simulink model "Control"  (R2023b)
settings: Solver=VariableStepAuto  StartTime=0.0  StopTime=0.5  RelTol=1e-3
values from neighbouring files (symbols this model uses):
  f_v = 1.7086e-04    (= 0.00017086)    [Control0.m]
  i = 12    [Control0.m]    (also in Electromechanical_coupling0.m; Figure3_9.m; Figure4_1819.m)
  J = J_m+J_eq+J_L/(i^2)    (= 0.000140202493333)    [Control0.m]    (also in Electromechanical_coupling0.m; Figure3_9.m = 0.000114299715556)
  J_eq = 3.53416e-6    (= 3.53416e-06)    [Control0.m]    (also in Electromechanical_coupling0.m)
  J_L = 4530e-6    (= 0.00453)    [Control0.m]    (also in Electromechanical_coupling0.m)
  J_m = 105.21e-6    (= 0.00010521)    [Control0.m]    (also in Electromechanical_coupling0.m)
  J_total = J_m+J_eq+(1/(i^2)+miu/i)*J_L    (= 0.000143184743333)    [Control0.m]
  Jeq = 3.53416e-6    (= 3.53416e-06)    [Figure3_9.m]    (also in Figure4_1819.m = 0.000143184743333)
  JL = 800e-6    (= 0.0008)    [Figure3_9.m]    (also in Figure4_1819.m = 0.00453)
  Jm = 105.21e-6    (= 0.00010521)    [Figure3_9.m]    (also in Figure4_1819.m)
  K_t = 3/2 * P_n * phi_f    (= 0.28077)    [Control0.m]    (also in Electromechanical_coupling0.m)
  Kic = 2000    [Control0.m]    (also in Figure3_9.m)
  Kic_2 = R_s/L_q    (= 719.178082192)    [Control0.m]
  Kis = 10    [Control0.m]    (also in Figure3_9.m = 20)
  Kis_2 = 1/(3*TPWM*delta^2)    (= 92.5925925926)    [Control0.m]
  Kpc = 3    [Control0.m]    (also in Figure3_9.m)
  Kpc_2 = L_q/(3*TPWM)    (= 4.86666666667)    [Control0.m]
  Kps = 0.15    [Control0.m]    (also in Figure3_9.m = 0.2)
  Kps_2 = J_total/(3*TPWM*delta*K_t)    (= 0.283317589592)    [Control0.m]
  Kt = 3/2 * Pn * Flux    (= 0.28077)    [Figure3_9.m]    (also in Figure4_1819.m)
  L_d = 1.46e-3    (= 0.00146)    [Control0.m]    (also in Electromechanical_coupling0.m)
  L_q = L_d    (= 0.00146)    [Control0.m]    (also in Electromechanical_coupling0.m)
  miu = 0.0079    [Control0.m]    (also in Figure4_1819.m)
  NtoW = pi / 30    (= 0.10471975512)    [Control0.m]    (also in Electromechanical_coupling0.m)
  P_n = 14    [Control0.m]    (also in Electromechanical_coupling0.m)
  phi_f = 0.01337    [Control0.m]    (also in Electromechanical_coupling0.m)
  R_s = 1.05    [Control0.m]    (also in Electromechanical_coupling0.m)
  T_c0 = 0.0104    [Control0.m]
  TPWM = 1/10000    (= 0.0001)    [Control0.m]
  U_dc = 72    [Control0.m]
  WtoN = 30 / pi    (= 9.54929658551)    [Control0.m]    (also in Electromechanical_coupling0.m)
undefined symbols (not defined in the file or in its folder): fv, Tc0
libraries: spsStairGeneratorLib x20, slpidlib x15, spsDCVoltageSourceLib x5, spsUniversalBridgeLib x5, spsPermanentMagnetSynchronousMachineLib x5, spsSVPWMGenerator2LevelLib x5, sps_lib x1, simulink x1
(part 1 of 3)
settings Model: Creator=Administrator  LastModifiedBy=Administrator

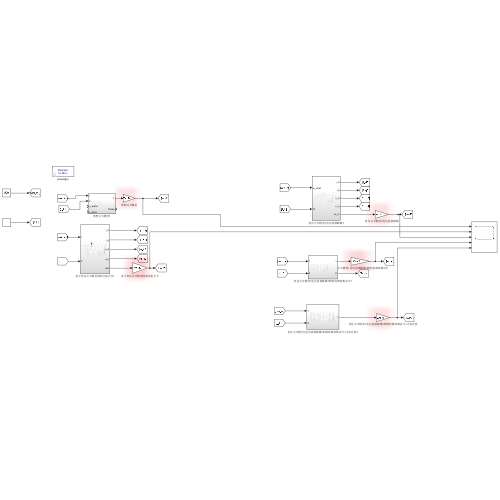
[thumbnail: Simulink's stored preview of the top-level diagram]
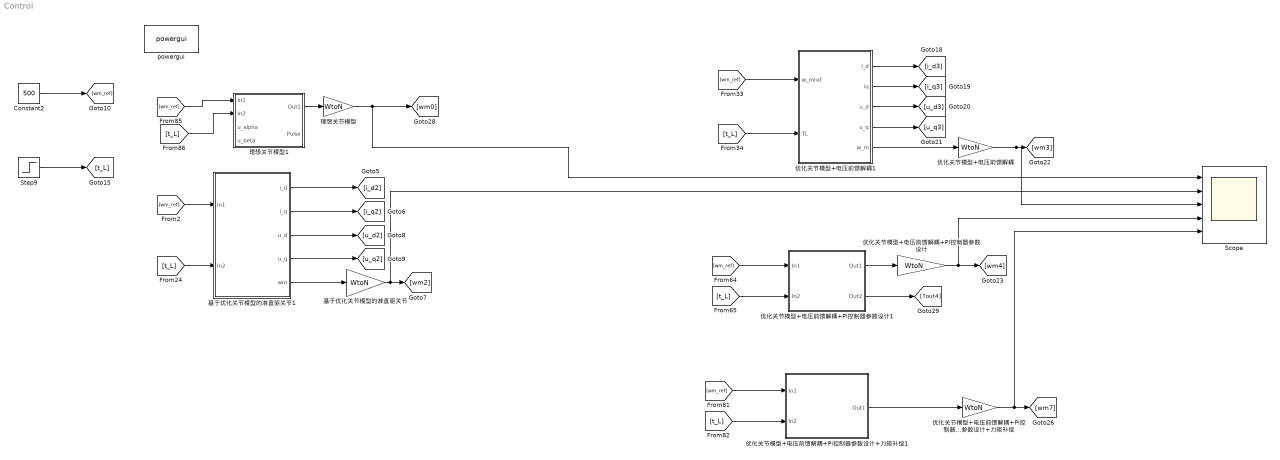
== system Control ==
  Constant2 : Constant  Value=500  SampleTime=-1
  Scope : Scope  NumInputPorts=5
  Step9 : Step  Time=0.2  After=3  SampleTime=0
  powergui : sps_lib/powergui  Priority=1  SimulationMode=Discrete  SampleTime=1e-6  frequency=60  Iterations=50  frequencyindice=0  Pbase=100e6  ErrMax=1e-4  UnitsV=kV  UnitsW=MW  buscounter=0  FunctionMessages=off  echomessages=off  EnableUseOfTLC=off  CurrentSourceSwitches=off  DisableSnubberDevices=off  DisableRonSwitches=off  DisableVfSwitches=off  DisplayEquations=off  AutomaticDiscreteSolvers=off  SolverType=Tustin/Backward Euler (TBE)  Interpol=off  ExternalGateDelay=off  methode=off  Ts=100  x0status=blocks  SPID=on  SwTol=0  HookPort=off  NonlinearTolerance=1e-4  nMaxIteration=100  ContinueOnMaxIteration=off  RestoreLinks=warning  ResistiveCurrentMeasurement=off  Frange=[0:2:500]  Ylog=off  Xlog=on  ShowGrid=off  save=off  variable=ZData  structure=0  ZoomFFT=off  StartTime=0.0  cycles=1  DisplayStyle=1  fundamental=60  FreqAxis=off  MaxFrequency=1000  frequencyindicesteady=1  RmsSteady=1  display=off
  优化关节模型+电压前馈解耦 : Gain  Gain=WtoN
  优化关节模型+电压前馈解耦+PI控制器参数设计 : Gain  Gain=WtoN
  优化关节模型+电压前馈解耦+PI控制器参数设计+力矩补偿 : Gain  Gain=WtoN
  优化关节模型+电压前馈解耦+PI控制器参数设计+力矩补偿1 : Subsystem
  优化关节模型+电压前馈解耦+PI控制器参数设计1 : Subsystem
  优化关节模型+电压前馈解耦1 : Subsystem
  基于优化关节模型的准直驱关节 : Gain  Gain=WtoN
  基于优化关节模型的准直驱关节1 : Subsystem
  理想关节模型 : Gain  Gain=WtoN
  理想关节模型1 : Subsystem
  wires:
  [t_L] -> 理想关节模型1/2(In2)
  [wm_ref] -> 理想关节模型1/1(In1)
  理想关节模型1/1(Out1) -> 理想关节模型/1
  Step9/1 -> [t_L]
  Constant2/1 -> [wm_ref]
  理想关节模型/1 -> Scope/1, [wm0]
  基于优化关节模型的准直驱关节1/5(wm) -> 基于优化关节模型的准直驱关节/1
  [wm_ref] -> 基于优化关节模型的准直驱关节1/1(In1)
  基于优化关节模型的准直驱关节1/1(i_d) -> [i_d2]
  基于优化关节模型的准直驱关节1/4(u_q) -> [u_q2]
  基于优化关节模型的准直驱关节1/2(i_q) -> [i_q2]
  [t_L] -> 基于优化关节模型的准直驱关节1/2(In2)
  基于优化关节模型的准直驱关节1/3(u_d) -> [u_d2]
  基于优化关节模型的准直驱关节/1 -> Scope/2, [wm2]
  优化关节模型+电压前馈解耦1/5(w_m) -> 优化关节模型+电压前馈解耦/1
  优化关节模型+电压前馈解耦1/3(u_d) -> [u_d3]
  优化关节模型+电压前馈解耦1/2(iq) -> [i_q3]
  优化关节模型+电压前馈解耦1/4(u_q) -> [u_q3]
  优化关节模型+电压前馈解耦1/1(i_d) -> [i_d3]
  [wm_ref] -> 优化关节模型+电压前馈解耦1/1(w_mref)
  [t_L] -> 优化关节模型+电压前馈解耦1/2(TL)
  优化关节模型+电压前馈解耦/1 -> [wm3], Scope/3
  [wm_ref] -> 优化关节模型+电压前馈解耦+PI控制器参数设计1/1(In1)
  优化关节模型+电压前馈解耦+PI控制器参数设计1/1(Out1) -> 优化关节模型+电压前馈解耦+PI控制器参数设计/1
  [t_L] -> 优化关节模型+电压前馈解耦+PI控制器参数设计1/2(In2)
  优化关节模型+电压前馈解耦+PI控制器参数设计1/2(Out2) -> [Tout4]
  优化关节模型+电压前馈解耦+PI控制器参数设计/1 -> Scope/4, [wm4]
  [t_L] -> 优化关节模型+电压前馈解耦+PI控制器参数设计+力矩补偿1/2(In2)
  [wm_ref] -> 优化关节模型+电压前馈解耦+PI控制器参数设计+力矩补偿1/1(In1)
  优化关节模型+电压前馈解耦+PI控制器参数设计+力矩补偿1/1(Out1) -> 优化关节模型+电压前馈解耦+PI控制器参数设计+力矩补偿/1
  优化关节模型+电压前馈解耦+PI控制器参数设计+力矩补偿/1 -> Scope/5, [wm7]

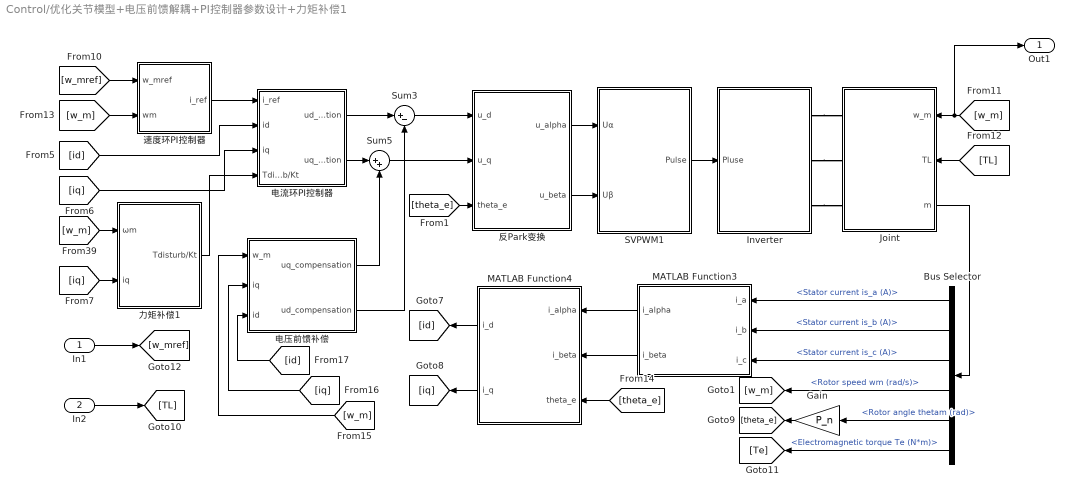
== system Control/优化关节模型+电压前馈解耦+PI控制器参数设计+力矩补偿1 ==
  In1 : Inport
  In2 : Inport  Port=2
  Bus Selector : BusSelector  OutputSignals=Stator current is_a (A),Stator current is_b (A),Stator current is_c (A),Rotor speed wm (rad/s),Rotor angle thetam (rad),Electromagnetic torque Te (N*m)
  Gain : Gain  Gain=P_n
  Inverter : Subsystem
  Joint : Subsystem
      settings: PortSchema="{\"entries\":[{\"content\":{\"sides\":[{\"content\":{\"connectorIds\":[\"LConn1\",\"LConn2\",\"LConn3\"]},\"type\":\"ConnectorPlacement.EquallySpacedRectSide\",\"uuid\":\"26e0b6e7-0d54-4404-9547-0f1b410a8b1d\"},{\"content\":{\"connectorIds\":[\"In1\",\"In2\",\"Out1\"],\"side\":\"RIGHT\"},\"type\":\"ConnectorPlacement.EquallySpacedRectSide\",\"uuid\":\"b2a73b6b-fc12-46f8-b2bb-dde1b38e1ce2\"},{\"content\":{\"side\":\"TOP\"},\"type\":\"ConnectorPlacement.EquallySpacedRectSide\",\"uuid\":\"06671ce4-b326-405e-8fb8-0b967c38d7ba\"}]},\"type\":\"ConnectorPlacement.EquallySpacedConnector\",\"uuid\":\"b49e6c2f-5ca5-4a6f-a472-6cb3ae827159\"}],\"packageUris\":[\"http://schema.mathworks.com/mf0/Connector/R2020b\"],\"version\":\"1.0\"}"
  MATLAB Function3 : MATLAB Function  TreatAsAtomicUnit=on
  MATLAB Function4 : MATLAB Function  TreatAsAtomicUnit=on
  SVPWM1 : Subsystem
  Sum3 : Sum  Inputs=|+-
  Sum5 : Sum  Inputs=|++
  力矩补偿1 : Subsystem
  反Park变换 : MATLAB Function  TreatAsAtomicUnit=on
  电压前馈补偿 : Subsystem
  电流环PI控制器 : Subsystem
  速度环PI控制器 : Subsystem
  Out1 : Outport
  wires:
  [w_m] -> Joint/1(w_m), Out1/1
  [w_m] -> 力矩补偿1/1(ωm)
  Gain/1 -> [theta_e]
  [theta_e] -> 反Park变换/3(theta_e)
  反Park变换/2(u_beta) -> SVPWM1/2(Uβ)
  [theta_e] -> MATLAB Function4/3(theta_e)
  MATLAB Function3/2(i_beta) -> MATLAB Function4/2(i_beta)
  Bus Selector/6 -> [Te]  "<Electromagnetic torque Te (N*m)>"
  [iq] -> 电压前馈补偿/2(iq)
  Bus Selector/4 -> [w_m]  "<Rotor speed wm (rad/s)>"
  Joint/1(m) -> Bus Selector/1
  [TL] -> Joint/2(TL)
  Bus Selector/5 -> Gain/1  "<Rotor angle thetam (rad)>"
  [id] -> 电压前馈补偿/3(id)
  In1/1 -> [w_mref]
  In2/1 -> [TL]
  SVPWM1/1(Pulse) -> Inverter/1(Pluse)
  Bus Selector/1 -> MATLAB Function3/1(i_a)  "<Stator current is_a (A)>"
  [w_m] -> 速度环PI控制器/2(wm)
  速度环PI控制器/1(i_ref) -> 电流环PI控制器/1(i_ref)
  MATLAB Function3/1(i_alpha) -> MATLAB Function4/1(i_alpha)
  [w_mref] -> 速度环PI控制器/1(w_mref)
  [w_m] -> 电压前馈补偿/1(w_m)
  [id] -> 电流环PI控制器/2(id)
  [iq] -> 电流环PI控制器/3(iq)
  电流环PI控制器/2(uq_equation) -> Sum5/1
  Bus Selector/2 -> MATLAB Function3/2(i_b)  "<Stator current is_b (A)>"
  Sum3/1 -> 反Park变换/1(u_d)
  Sum5/1 -> 反Park变换/2(u_q)
  电流环PI控制器/1(ud_equation) -> Sum3/1
  Bus Selector/3 -> MATLAB Function3/3(i_c)  "<Stator current is_c (A)>"
  反Park变换/1(u_alpha) -> SVPWM1/1(Uα)
  [iq] -> 力矩补偿1/2(iq)
  力矩补偿1/1(Tdisturb/Kt) -> 电流环PI控制器/4(Tdisturb/Kt)
  MATLAB Function4/1(i_d) -> [id]
  MATLAB Function4/2(i_q) -> [iq]
  电压前馈补偿/1(uq_compensation) -> Sum5/2
  电压前馈补偿/2(ud_compensation) -> Sum3/2
  connections:
  Inverter/RConn1 -- Joint/LConn1
  Inverter/RConn2 -- Joint/LConn2
  Inverter/RConn3 -- Joint/LConn3

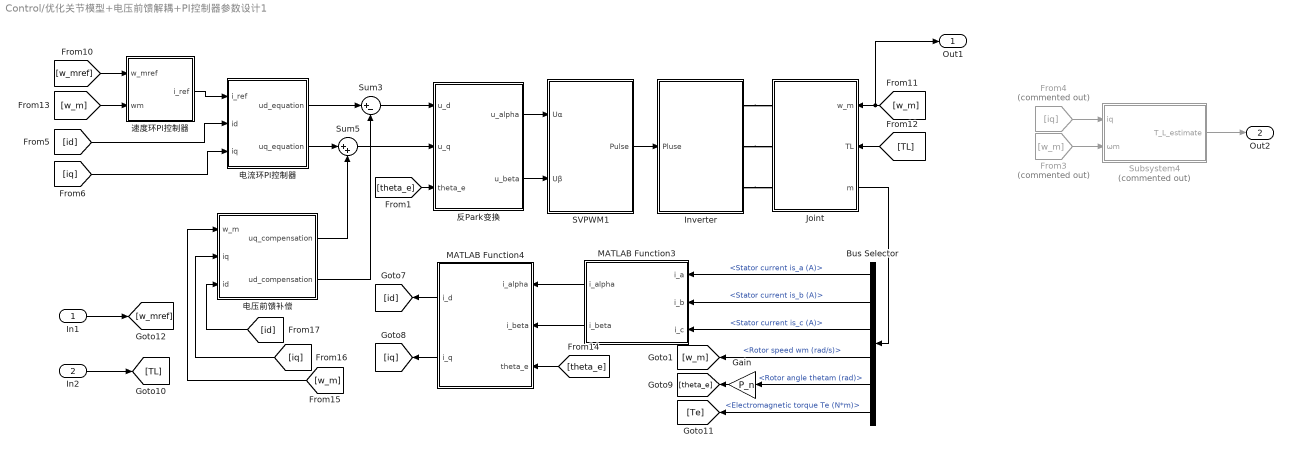
== system Control/优化关节模型+电压前馈解耦+PI控制器参数设计1 ==
  In1 : Inport
  In2 : Inport  Port=2
  Bus Selector : BusSelector  OutputSignals=Stator current is_a (A),Stator current is_b (A),Stator current is_c (A),Rotor speed wm (rad/s),Rotor angle thetam (rad),Electromagnetic torque Te (N*m)
  From3 : From  Commented=on  GotoTag=w_m
  From4 : From  Commented=on  GotoTag=iq
  Gain : Gain  Gain=P_n
  Inverter : Subsystem
  Joint : Subsystem
      settings: PortSchema="{\"entries\":[{\"content\":{\"sides\":[{\"content\":{\"connectorIds\":[\"LConn1\",\"LConn2\",\"LConn3\"]},\"type\":\"ConnectorPlacement.EquallySpacedRectSide\",\"uuid\":\"26e0b6e7-0d54-4404-9547-0f1b410a8b1d\"},{\"content\":{\"connectorIds\":[\"In1\",\"In2\",\"Out1\"],\"side\":\"RIGHT\"},\"type\":\"ConnectorPlacement.EquallySpacedRectSide\",\"uuid\":\"b2a73b6b-fc12-46f8-b2bb-dde1b38e1ce2\"},{\"content\":{\"side\":\"TOP\"},\"type\":\"ConnectorPlacement.EquallySpacedRectSide\",\"uuid\":\"06671ce4-b326-405e-8fb8-0b967c38d7ba\"}]},\"type\":\"ConnectorPlacement.EquallySpacedConnector\",\"uuid\":\"b49e6c2f-5ca5-4a6f-a472-6cb3ae827159\"}],\"packageUris\":[\"http://schema.mathworks.com/mf0/Connector/R2020b\"],\"version\":\"1.0\"}"
  MATLAB Function3 : MATLAB Function  TreatAsAtomicUnit=on
  MATLAB Function4 : MATLAB Function  TreatAsAtomicUnit=on
  SVPWM1 : Subsystem
  Subsystem4 : Subsystem  Commented=on
  Sum3 : Sum  Inputs=|+-
  Sum5 : Sum  Inputs=|++
  反Park变换 : MATLAB Function  TreatAsAtomicUnit=on
  电压前馈补偿 : Subsystem
  电流环PI控制器 : Subsystem
  速度环PI控制器 : Subsystem
  Out1 : Outport
  Out2 : Outport  Port=2
  wires:
  电压前馈补偿/2(ud_compensation) -> Sum3/2
  电压前馈补偿/1(uq_compensation) -> Sum5/2
  MATLAB Function4/2(i_q) -> [iq]
  MATLAB Function4/1(i_d) -> [id]
  反Park变换/1(u_alpha) -> SVPWM1/1(Uα)
  Bus Selector/3 -> MATLAB Function3/3(i_c)  "<Stator current is_c (A)>"
  电流环PI控制器/1(ud_equation) -> Sum3/1
  Sum5/1 -> 反Park变换/2(u_q)
  Sum3/1 -> 反Park变换/1(u_d)
  Bus Selector/2 -> MATLAB Function3/2(i_b)  "<Stator current is_b (A)>"
  电流环PI控制器/2(uq_equation) -> Sum5/1
  [iq] -> 电流环PI控制器/3(iq)
  [id] -> 电流环PI控制器/2(id)
  [w_m] -> 电压前馈补偿/1(w_m)
  [w_mref] -> 速度环PI控制器/1(w_mref)
  MATLAB Function3/1(i_alpha) -> MATLAB Function4/1(i_alpha)
  速度环PI控制器/1(i_ref) -> 电流环PI控制器/1(i_ref)
  [w_m] -> 速度环PI控制器/2(wm)
  Bus Selector/1 -> MATLAB Function3/1(i_a)  "<Stator current is_a (A)>"
  SVPWM1/1(Pulse) -> Inverter/1(Pluse)
  In2/1 -> [TL]
  In1/1 -> [w_mref]
  [id] -> 电压前馈补偿/3(id)
  Bus Selector/5 -> Gain/1  "<Rotor angle thetam (rad)>"
  [TL] -> Joint/2(TL)
  Joint/1(m) -> Bus Selector/1
  Bus Selector/4 -> [w_m]  "<Rotor speed wm (rad/s)>"
  [iq] -> 电压前馈补偿/2(iq)
  Bus Selector/6 -> [Te]  "<Electromagnetic torque Te (N*m)>"
  MATLAB Function3/2(i_beta) -> MATLAB Function4/2(i_beta)
  [theta_e] -> MATLAB Function4/3(theta_e)
  反Park变换/2(u_beta) -> SVPWM1/2(Uβ)
  [theta_e] -> 反Park变换/3(theta_e)
  Gain/1 -> [theta_e]
  [w_m] -> Out1/1, Joint/1(w_m)
  Subsystem4/1(T_L_estimate) -> Out2/1
  From4/1 -> Subsystem4/1(iq)
  From3/1 -> Subsystem4/2(ωm)
  connections:
  Inverter/RConn3 -- Joint/LConn3
  Inverter/RConn2 -- Joint/LConn2
  Inverter/RConn1 -- Joint/LConn1

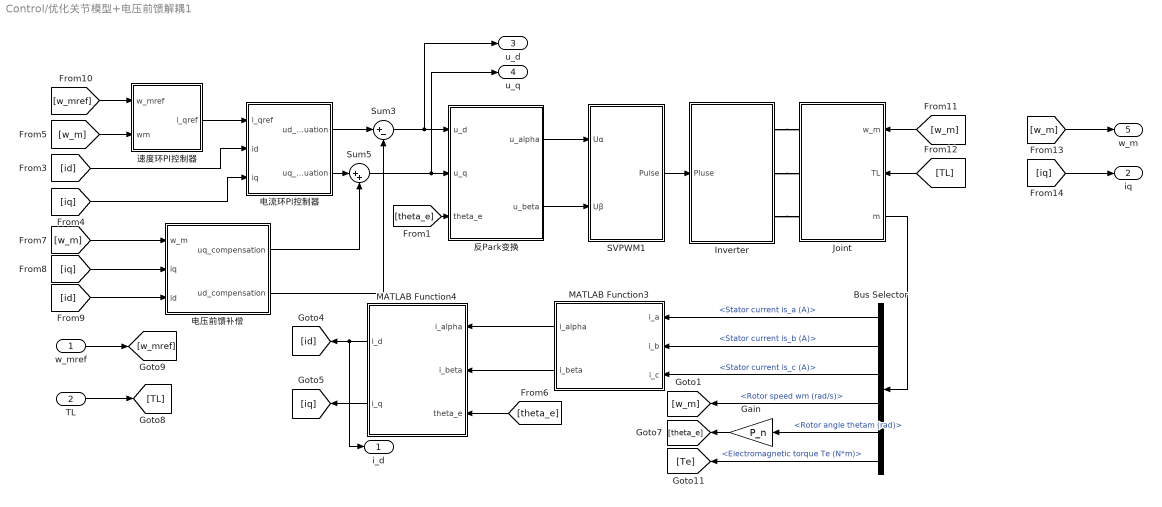
== system Control/优化关节模型+电压前馈解耦1 ==
  w_mref : Inport
  TL : Inport  Port=2
  Bus Selector : BusSelector  OutputSignals=Stator current is_a (A),Stator current is_b (A),Stator current is_c (A),Rotor speed wm (rad/s),Rotor angle thetam (rad),Electromagnetic torque Te (N*m)
  Gain : Gain  Gain=P_n
  Inverter : Subsystem
  Joint : Subsystem
      settings: PortSchema="{\"entries\":[{\"content\":{\"sides\":[{\"content\":{\"connectorIds\":[\"LConn1\",\"LConn2\",\"LConn3\"]},\"type\":\"ConnectorPlacement.EquallySpacedRectSide\",\"uuid\":\"26e0b6e7-0d54-4404-9547-0f1b410a8b1d\"},{\"content\":{\"connectorIds\":[\"In1\",\"In2\",\"Out1\"],\"side\":\"RIGHT\"},\"type\":\"ConnectorPlacement.EquallySpacedRectSide\",\"uuid\":\"b2a73b6b-fc12-46f8-b2bb-dde1b38e1ce2\"},{\"content\":{\"side\":\"TOP\"},\"type\":\"ConnectorPlacement.EquallySpacedRectSide\",\"uuid\":\"06671ce4-b326-405e-8fb8-0b967c38d7ba\"}]},\"type\":\"ConnectorPlacement.EquallySpacedConnector\",\"uuid\":\"b49e6c2f-5ca5-4a6f-a472-6cb3ae827159\"}],\"packageUris\":[\"http://schema.mathworks.com/mf0/Connector/R2020b\"],\"version\":\"1.0\"}"
  MATLAB Function3 : MATLAB Function  TreatAsAtomicUnit=on
  MATLAB Function4 : MATLAB Function  TreatAsAtomicUnit=on
  SVPWM1 : Subsystem
  Sum3 : Sum  Inputs=|+-
  Sum5 : Sum  Inputs=|++
  反Park变换 : MATLAB Function  TreatAsAtomicUnit=on
  电压前馈补偿 : Subsystem
  电流环PI控制器 : Subsystem
  速度环PI控制器 : Subsystem
  i_d : Outport
  iq : Outport  Port=2
  u_d : Outport  Port=3
  u_q : Outport  Port=4
  w_m : Outport  Port=5
  wires:
  w_mref/1 -> [w_mref]
  Sum3/1 -> u_d/1, 反Park变换/1(u_d)
  Sum5/1 -> 反Park变换/2(u_q), u_q/1
  [iq] -> 电流环PI控制器/3(iq)
  [w_mref] -> 速度环PI控制器/1(w_mref)
  [theta_e] -> MATLAB Function4/3(theta_e)
  [w_m] -> 速度环PI控制器/2(wm)
  MATLAB Function4/2(i_q) -> [iq]
  Bus Selector/2 -> MATLAB Function3/2(i_b)  "<Stator current is_b (A)>"
  速度环PI控制器/1(i_qref) -> 电流环PI控制器/1(i_qref)
  电流环PI控制器/1(ud_equation) -> Sum3/1
  反Park变换/2(u_beta) -> SVPWM1/2(Uβ)
  [id] -> 电流环PI控制器/2(id)
  MATLAB Function3/2(i_beta) -> MATLAB Function4/2(i_beta)
  Bus Selector/1 -> MATLAB Function3/1(i_a)  "<Stator current is_a (A)>"
  MATLAB Function3/1(i_alpha) -> MATLAB Function4/1(i_alpha)
  Gain/1 -> [theta_e]
  Bus Selector/4 -> [w_m]  "<Rotor speed wm (rad/s)>"
  Bus Selector/6 -> [Te]  "<Electromagnetic torque Te (N*m)>"
  SVPWM1/1(Pulse) -> Inverter/1(Pluse)
  Bus Selector/3 -> MATLAB Function3/3(i_c)  "<Stator current is_c (A)>"
  [theta_e] -> 反Park变换/3(theta_e)
  [iq] -> 电压前馈补偿/2(iq)
  MATLAB Function4/1(i_d) -> i_d/1, [id]
  Bus Selector/5 -> Gain/1  "<Rotor angle thetam (rad)>"
  [id] -> 电压前馈补偿/3(id)
  [w_m] -> Joint/1(w_m)
  [TL] -> Joint/2(TL)
  Joint/1(m) -> Bus Selector/1
  [w_m] -> 电压前馈补偿/1(w_m)
  TL/1 -> [TL]
  [w_m] -> w_m/1
  [iq] -> iq/1
  反Park变换/1(u_alpha) -> SVPWM1/1(Uα)
  电流环PI控制器/2(uq_equation) -> Sum5/1
  电压前馈补偿/1(uq_compensation) -> Sum5/2
  电压前馈补偿/2(ud_compensation) -> Sum3/2
  connections:
  Inverter/RConn3 -- Joint/LConn3
  Inverter/RConn2 -- Joint/LConn2
  Inverter/RConn1 -- Joint/LConn1

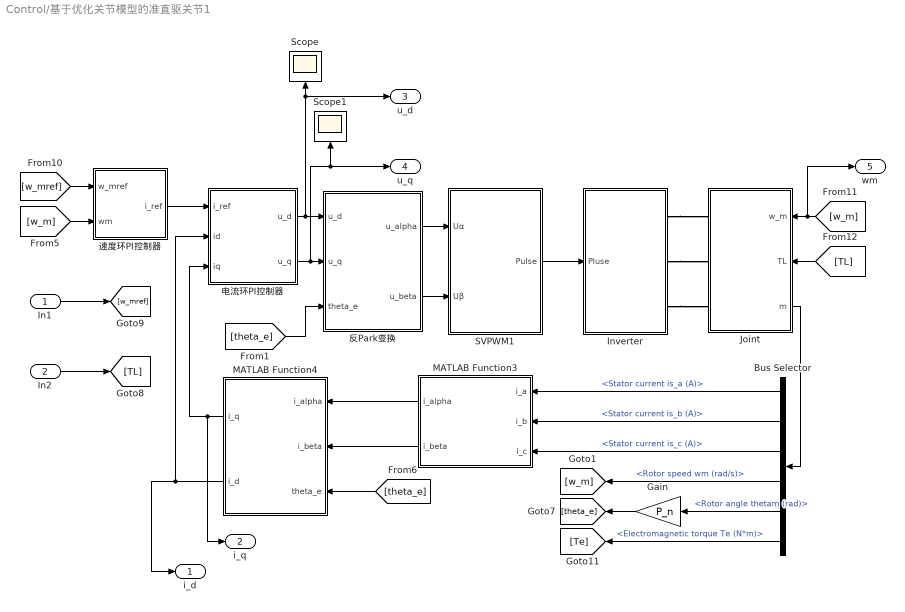
== system Control/基于优化关节模型的准直驱关节1 ==
  In1 : Inport
  In2 : Inport  Port=2
  Bus Selector : BusSelector  OutputSignals=Stator current is_a (A),Stator current is_b (A),Stator current is_c (A),Rotor speed wm (rad/s),Rotor angle thetam (rad),Electromagnetic torque Te (N*m)
  Gain : Gain  Gain=P_n
  Inverter : Subsystem
  Joint : Subsystem
      settings: PortSchema="{\"entries\":[{\"content\":{\"sides\":[{\"content\":{\"connectorIds\":[\"LConn1\",\"LConn2\",\"LConn3\"]},\"type\":\"ConnectorPlacement.EquallySpacedRectSide\",\"uuid\":\"26e0b6e7-0d54-4404-9547-0f1b410a8b1d\"},{\"content\":{\"connectorIds\":[\"In1\",\"In2\",\"Out1\"],\"side\":\"RIGHT\"},\"type\":\"ConnectorPlacement.EquallySpacedRectSide\",\"uuid\":\"b2a73b6b-fc12-46f8-b2bb-dde1b38e1ce2\"},{\"content\":{\"side\":\"TOP\"},\"type\":\"ConnectorPlacement.EquallySpacedRectSide\",\"uuid\":\"06671ce4-b326-405e-8fb8-0b967c38d7ba\"}]},\"type\":\"ConnectorPlacement.EquallySpacedConnector\",\"uuid\":\"b49e6c2f-5ca5-4a6f-a472-6cb3ae827159\"}],\"packageUris\":[\"http://schema.mathworks.com/mf0/Connector/R2020b\"],\"version\":\"1.0\"}"
  MATLAB Function3 : MATLAB Function  TreatAsAtomicUnit=on
  MATLAB Function4 : MATLAB Function  TreatAsAtomicUnit=on
  SVPWM1 : Subsystem
  Scope : Scope
  Scope1 : Scope
  反Park变换 : MATLAB Function  TreatAsAtomicUnit=on
  电流环PI控制器 : Subsystem
  速度环PI控制器 : Subsystem
  i_d : Outport
  i_q : Outport  Port=2
  u_d : Outport  Port=3
  u_q : Outport  Port=4
  wm : Outport  Port=5
  wires:
  In2/1 -> [TL]
  In1/1 -> [w_mref]
  [TL] -> Joint/2(TL)
  Bus Selector/5 -> Gain/1  "<Rotor angle thetam (rad)>"
  Bus Selector/1 -> MATLAB Function3/1(i_a)  "<Stator current is_a (A)>"
  Joint/1(m) -> Bus Selector/1
  Bus Selector/4 -> [w_m]  "<Rotor speed wm (rad/s)>"
  [theta_e] -> 反Park变换/3(theta_e)
  Bus Selector/3 -> MATLAB Function3/3(i_c)  "<Stator current is_c (A)>"
  Bus Selector/6 -> [Te]  "<Electromagnetic torque Te (N*m)>"
  SVPWM1/1(Pulse) -> Inverter/1(Pluse)
  Gain/1 -> [theta_e]
  MATLAB Function3/2(i_beta) -> MATLAB Function4/2(i_beta)
  [theta_e] -> MATLAB Function4/3(theta_e)
  MATLAB Function3/1(i_alpha) -> MATLAB Function4/1(i_alpha)
  反Park变换/1(u_alpha) -> SVPWM1/1(Uα)
  反Park变换/2(u_beta) -> SVPWM1/2(Uβ)
  电流环PI控制器/2(u_q) -> u_q/1, Scope1/1, 反Park变换/2(u_q)
  [w_m] -> 速度环PI控制器/2(wm)
  速度环PI控制器/1(i_ref) -> 电流环PI控制器/1(i_ref)
  [w_mref] -> 速度环PI控制器/1(w_mref)
  Bus Selector/2 -> MATLAB Function3/2(i_b)  "<Stator current is_b (A)>"
  MATLAB Function4/2(i_d) -> i_d/1, 电流环PI控制器/2(id)
  MATLAB Function4/1(i_q) -> i_q/1, 电流环PI控制器/3(iq)
  [w_m] -> wm/1, Joint/1(w_m)
  电流环PI控制器/1(u_d) -> u_d/1, Scope/1, 反Park变换/1(u_d)
  connections:
  Inverter/RConn1 -- Joint/LConn1
  Inverter/RConn3 -- Joint/LConn3
  Inverter/RConn2 -- Joint/LConn2

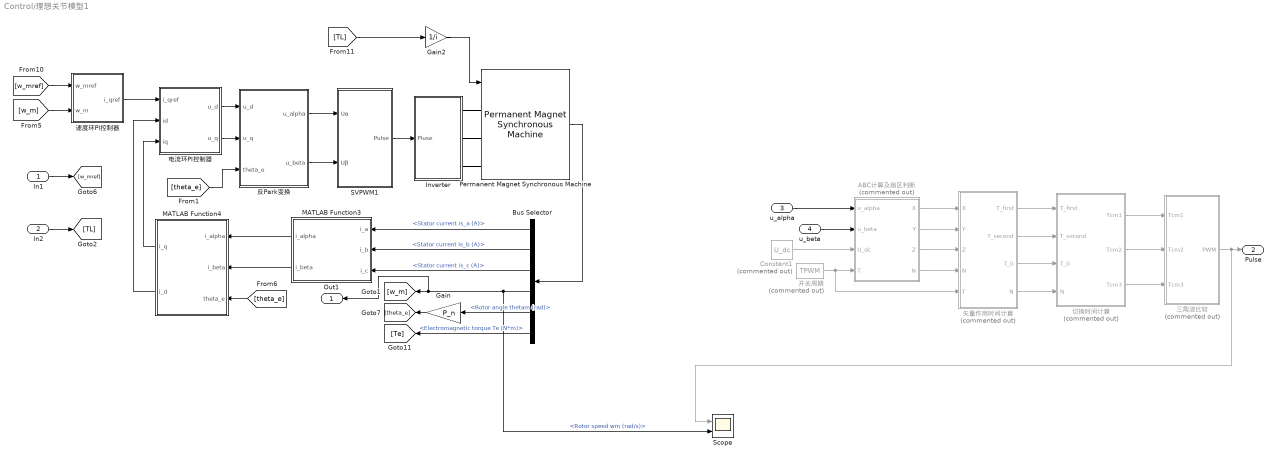
== system Control/理想关节模型1 ==
  In1 : Inport
  In2 : Inport  Port=2
  u_alpha : Inport  Port=3
  u_beta : Inport  Port=4
  ABC计算及扇区判断 : MATLAB Function  Commented=on  TreatAsAtomicUnit=on
  Bus Selector : BusSelector  OutputSignals=Stator current is_a (A),Stator current is_b (A),Stator current is_c (A),Rotor speed wm (rad/s),Rotor angle thetam (rad),Electromagnetic torque Te (N*m)
  Constant1 : Constant  Commented=on  Value=U_dc  SampleTime=-1
  Gain : Gain  Gain=P_n
  Gain2 : Gain  Gain=1/i
  Inverter : Subsystem
  MATLAB Function3 : MATLAB Function  TreatAsAtomicUnit=on
  MATLAB Function4 : MATLAB Function  TreatAsAtomicUnit=on
  Permanent Magnet Synchronous Machine : spsPermanentMagnetSynchronousMachineLib/Permanent Magnet Synchronous Machine  NbPhases=3  FluxDistribution=Sinusoidal  RotorType=Round  MechanicalLoad=Torque Tm  PresetModel=No  ShowDetailedParameters=on  MeasurementBus=off  Resistance=R_s  Inductance=8.5e-3  dqInductances=[2.27e-3,2.045e-3]  La=L_q  MachineConstant=Torque Constant (N.m / A_peak)  Flux=0.046795  VoltageCst=33.9507  TorqueCst=K_t  Flat=120  Mechanical=[J 0 P_n 0]  PolePairs=4  InitialConditions=[0,0, 0,0]  InitialConditions5ph=[0 0 0 0 0 0]  RefAngle=Aligned with phase A axis (original Park)  IterativeDiscreteModel=Trapezoidal non iterative  TsBlock=-1  TsPowergui=0
  SVPWM1 : Subsystem
  Scope : Scope  NumInputPorts=2
  三角波比较 : Subsystem  Commented=on
  切换时间计算 : MATLAB Function  Commented=on  TreatAsAtomicUnit=on
  反Park变换 : MATLAB Function  TreatAsAtomicUnit=on
  开关周期 : Constant  Commented=on  Value=TPWM  SampleTime=-1
  电流环PI控制器 : Subsystem
  矢量作用时间计算 : MATLAB Function  Commented=on  TreatAsAtomicUnit=on
  速度环PI控制器 : Subsystem
  Out1 : Outport
  Pulse : Outport  Port=2
  wires:
  Bus Selector/5 -> Gain/1  "<Rotor angle thetam (rad)>"
  Bus Selector/1 -> MATLAB Function3/1(i_a)  "<Stator current is_a (A)>"
  Permanent Magnet Synchronous Machine/1 -> Bus Selector/1
  Bus Selector/4 -> Scope/2, Out1/1, [w_m]  "<Rotor speed wm (rad/s)>"
  [theta_e] -> 反Park变换/3(theta_e)
  Bus Selector/3 -> MATLAB Function3/3(i_c)  "<Stator current is_c (A)>"
  Bus Selector/6 -> [Te]  "<Electromagnetic torque Te (N*m)>"
  SVPWM1/1(Pulse) -> Inverter/1(Pluse)
  Gain/1 -> [theta_e]
  MATLAB Function3/2(i_beta) -> MATLAB Function4/2(i_beta)
  [theta_e] -> MATLAB Function4/3(theta_e)
  MATLAB Function3/1(i_alpha) -> MATLAB Function4/1(i_alpha)
  反Park变换/1(u_alpha) -> SVPWM1/1(Uα)
  反Park变换/2(u_beta) -> SVPWM1/2(Uβ)
  电流环PI控制器/2(u_q) -> 反Park变换/2(u_q)
  [w_m] -> 速度环PI控制器/2(w_m)
  速度环PI控制器/1(i_qref) -> 电流环PI控制器/1(i_qref)
  [w_mref] -> 速度环PI控制器/1(w_mref)
  Bus Selector/2 -> MATLAB Function3/2(i_b)  "<Stator current is_b (A)>"
  MATLAB Function4/2(i_d) -> 电流环PI控制器/2(id)
  MATLAB Function4/1(i_q) -> 电流环PI控制器/3(iq)
  Gain2/1 -> Permanent Magnet Synchronous Machine/1
  [TL] -> Gain2/1
  In1/1 -> [w_mref]
  In2/1 -> [TL]
  电流环PI控制器/1(u_d) -> 反Park变换/1(u_d)
  切换时间计算/1(Tcm1) -> 三角波比较/1(Tcm1)
  ABC计算及扇区判断/2(Y) -> 矢量作用时间计算/2(Y)
  ABC计算及扇区判断/4(N) -> 矢量作用时间计算/4("N ")
  矢量作用时间计算/1(T_first) -> 切换时间计算/1(T_first)
  开关周期/1 -> 矢量作用时间计算/5(T), ABC计算及扇区判断/4(T)
  三角波比较/1(PWM) -> Scope/1, Pulse/1
  切换时间计算/3(Tcm3) -> 三角波比较/3(Tcm3)
  矢量作用时间计算/2(T_second) -> 切换时间计算/2(T_second)
  ABC计算及扇区判断/3(Z) -> 矢量作用时间计算/3(Z)
  矢量作用时间计算/4(N) -> 切换时间计算/4(N)
  Constant1/1 -> ABC计算及扇区判断/3(U_dc)
  u_alpha/1 -> ABC计算及扇区判断/1(u_alpha)
  u_beta/1 -> ABC计算及扇区判断/2(u_beta)
  ABC计算及扇区判断/1(X) -> 矢量作用时间计算/1(X)
  矢量作用时间计算/3(T_0) -> 切换时间计算/3(T_0)
  切换时间计算/2(Tcm2) -> 三角波比较/2(Tcm2)
  connections:
  Permanent Magnet Synchronous Machine/LConn1 -- Inverter/RConn1
  Inverter/RConn3 -- Permanent Magnet Synchronous Machine/LConn3
  Permanent Magnet Synchronous Machine/LConn2 -- Inverter/RConn2

== system Control/优化关节模型+电压前馈解耦+PI控制器参数设计+力矩补偿1/Inverter ==
  Pluse : Inport
  DC Voltage Source1 : spsDCVoltageSourceLib/DC Voltage Source  Amplitude=U_dc  Measurements=None
  Universal Bridge : spsUniversalBridgeLib/Universal Bridge  Arms=3  SnubberResistance=1e5  SnubberCapacitance=inf  Device=IGBT / Diodes  Ron=1e-3  Lon=0  ForwardVoltages="[  0  0  ]"  ForwardVoltage=0  GTOparameters=[ 10e-6 , 20e-6 ]  IGBTparameters=[ 1e-6 , 2e-6 ]  Measurements=None  Measurements_2=None  converterType=Rectifier
  A : PMIOPort  Side=Right
  B : PMIOPort  Port=2  Side=Right
  C : PMIOPort  Port=3  Side=Right
  wires:
  Pluse/1 -> Universal Bridge/1
  connections:
  Universal Bridge/LConn2 -- B/RConn1
  DC Voltage Source1/RConn1 -- Universal Bridge/RConn1
  DC Voltage Source1/LConn1 -- Universal Bridge/RConn2
  Universal Bridge/LConn3 -- C/RConn1
  Universal Bridge/LConn1 -- A/RConn1

== system Control/优化关节模型+电压前馈解耦+PI控制器参数设计+力矩补偿1/Joint ==
  w_m : Inport
  TL : Inport  Port=2
  Permanent Magnet Synchronous Machine : spsPermanentMagnetSynchronousMachineLib/Permanent Magnet Synchronous Machine  NbPhases=3  FluxDistribution=Sinusoidal  RotorType=Round  MechanicalLoad=Torque Tm  PresetModel=No  ShowDetailedParameters=on  MeasurementBus=off  Resistance=R_s  Inductance=8.5e-3  dqInductances=[2.27e-3,2.045e-3]  La=L_q  MachineConstant=Torque Constant (N.m / A_peak)  Flux=0.01337  VoltageCst=33.9507  TorqueCst=K_t  Flat=120  Mechanical=[J_total 0 P_n 0]  PolePairs=4  InitialConditions=[0,0, 0,0]  InitialConditions5ph=[0 0 0 0 0 0]  RefAngle=Aligned with phase A axis (original Park)  IterativeDiscreteModel=Trapezoidal non iterative  TsBlock=-1  TsPowergui=0
  Subsystem : Subsystem
  A : PMIOPort  Side=Left
  B : PMIOPort  Port=2  Side=Left
  C : PMIOPort  Port=3  Side=Left
  m : Outport
  wires:
  TL/1 -> Subsystem/2(TL)
  Permanent Magnet Synchronous Machine/1 -> m/1
  Subsystem/1(Tm) -> Permanent Magnet Synchronous Machine/1
  w_m/1 -> Subsystem/1(wm)
  connections:
  A/RConn1 -- Permanent Magnet Synchronous Machine/LConn1
  B/RConn1 -- Permanent Magnet Synchronous Machine/LConn2
  C/RConn1 -- Permanent Magnet Synchronous Machine/LConn3

== system Control/优化关节模型+电压前馈解耦+PI控制器参数设计+力矩补偿1/SVPWM1 ==
  Uα : Inport
  Uβ : Inport  Port=2
  SVPWM Generator (2-Level) : spsSVPWMGenerator2LevelLib/SVPWM Generator (2-Level)  InputType=alpha-beta components  SwitchingPattern=Pattern #1  Fc=1/TPWM  ParUref=[0.8 -30 50]  Ts=0.000001
  Pulse : Outport
  wires:
  SVPWM Generator (2-Level)/1 -> Pulse/1
  Uα/1 -> SVPWM Generator (2-Level)/1
  Uβ/1 -> SVPWM Generator (2-Level)/2

== system Control/优化关节模型+电压前馈解耦+PI控制器参数设计+力矩补偿1/力矩补偿1 ==
  note: fv·ωm
  note: μ·TL·sgn(ωm)
  note: Tdisturb
  note: Tc0·sgn(ωm)
  note: sgn(ωm)
  ωm : Inport
  iq : Inport  Port=2
  Divide : Product  Inputs=**
  Gain : Gain  Gain=f_v
  Gain1 : Gain  Gain=T_c0
  Gain13 : Gain  Gain=miu
  Gain2 : Gain  Gain=1/K_t
  Load Torque (N.m)5 : spsStairGeneratorLib/Stair Generator  t=[0,0.308,0.614,0.939,1.273,1.587,1.902,2.259,2.564]  e=[9.97,15,20,24.7,22.3,20.3,18.7,17.3,16.1]  Ts=1e-6
  Scope : Scope
  Sign : Signum
  Subsystem4 : Subsystem
  Subtract : Sum  Inputs=+++
  Tdisturb/Kt : Outport
  wires:
  iq/1 -> Subsystem4/1(iq)
  Gain2/1 -> Tdisturb/Kt/1
  Gain/1 -> Subtract/3
  Divide/1 -> Subtract/1
  Gain1/1 -> Subtract/2
  ωm/1 -> Subsystem4/2(ωm), Gain/1, Sign/1
  Sign/1 -> Gain1/1, Divide/2
  Subtract/1 -> Gain2/1
  Subsystem4/1(T_L_estimate) -> Scope/1, Gain13/1
  Gain13/1 -> Divide/1

== system Control/优化关节模型+电压前馈解耦+PI控制器参数设计+力矩补偿1/电压前馈补偿 ==
  w_m : Inport
  iq : Inport  Port=2
  id : Inport  Port=3
  Add : Sum
  Constant2 : Constant  Value=phi_f
  Gain1 : Gain  Gain=L_d
  Gain2 : Gain  Gain=P_n
  Gain7 : Gain  Gain=L_q
  Product : Product
  Product1 : Product
  uq_compensation : Outport
  ud_compensation : Outport  Port=2
  wires:
  Constant2/1 -> Add/2
  Product1/1 -> uq_compensation/1
  id/1 -> Gain1/1
  Add/1 -> Product1/2
  Gain2/1 -> Product/1, Product1/1
  Gain1/1 -> Add/1
  Product/1 -> Gain7/1
  Gain7/1 -> ud_compensation/1
  iq/1 -> Product/2
  w_m/1 -> Gain2/1

== system Control/优化关节模型+电压前馈解耦+PI控制器参数设计+力矩补偿1/电流环PI控制器 ==
  note: uq_equation
  note: ud_equation
  i_ref : Inport
  id : Inport  Port=2
  iq : Inport  Port=3
  Tdisturb/Kt : Inport  Port=4
  Constant2 : Constant  Value=0
  PID Controller (2DOF)1 : slpidlib/PID Controller (2DOF)  Controller=PI  Form=Ideal  TimeDomain=Discrete-time  UseExternalTs=off  SampleTime=0.000001  IntegratorMethod=Forward Euler  FilterMethod=Forward Euler  ControllerParametersSource=internal  P=Kpc_2  I=Kic_2  UseKiTs=off  D=0  N=100  UseFilter=on  b=1  c=1  TunerSelectOption=Transfer Function Based (PID Tuner App)  InitialConditionSource=internal  InitialConditionForIntegrator=0  InitialConditionForFilter=0  DifferentiatorICPrevScaledInput=0  ExternalReset=none  TrackingMode=off  Kt=1  LimitOutput=on  SatLimitsSource=internal  UpperSaturationLimit=72/sqrt(3)  LowerSaturationLimit=-72/sqrt(3)  LinearizeAsGain=on  AntiWindupMode=none  Kb=1  LimitIntegrator=off  UpperIntegratorSaturationLimit=inf  LowerIntegratorSaturationLimit=-inf  POutMin=[]  POutMax=[]  IOutMin=[]  IOutMax=[]  DOutMin=[]  DOutMax=[]  NOutMin=[]  NOutMax=[]  bOutMin=[]  bOutMax=[]  cOutMin=[]  cOutMax=[]  SumOutMin=[]  SumOutMax=[]  SaturationOutMin=[]  SaturationOutMax=[]  PParamMin=[]  PParamMax=[]  IParamMin=[]  IParamMax=[]  DParamMin=[]  DParamMax=[]  NParamMin=[]  NParamMax=[]  bParamMin=[]  bParamMax=[]  cParamMin=[]  cParamMax=[]  KbParamMin=[]  KbParamMax=[]  KtParamMin=[]  KtParamMax=[]  KbOutMin=[]  KbOutMax=[]  KtOutMin=[]  KtOutMax=[]  IntegratorOutMin=[]  IntegratorOutMax=[]  FilterOutMin=[]  FilterOutMax=[]  SumI1OutMin=[]  SumI1OutMax=[]  SumI2OutMin=[]  SumI2OutMax=[]  SumI3OutMin=[]  SumI3OutMax=[]  SumI4OutMin=[]  SumI4OutMax=[]  SumDOutMin=[]  SumDOutMax=[]  Sum1OutMin=[]  Sum1OutMax=[]  Sum2OutMin=[]  Sum2OutMax=[]  Sum3OutMin=[]  Sum3OutMax=[]  DifferentiatorOutMin=[]  DifferentiatorOutMax=[]  FilterDiffOutCoefMin=[]  FilterDiffOutCoefMax=[]  ReciprocalOutMin=[]  ReciprocalOutMax=[]  SumDenOutMin=[]  SumDenOutMax=[]  SumNumOutMin=[]  SumNumOutMax=[]  DivideOutMin=[]  DivideOutMax=[]  UdiffTsProdOutMin=[]  UdiffTsProdOutMax=[]  NTsProdOutMin=[]  NTsProdOutMax=[]  UintegralTsProdOutMin=[]  UintegralTsProdOutMax=[]  UngainTsProdOutMin=[]  UngainTsProdOutMax=[]  ClampingZeroOutDataTypeStr=Inherit: Inherit via back propagation  ClampingZeroOutMin=[]  ClampingZeroOutMax=[]  FilterDenConstantOutDataTypeStr=Inherit: Inherit via back propagation  FilterDenConstantOutMin=[]  FilterDenConstantOutMax=[]  PCopyOutDataTypeStr=Inherit: Inherit via back propagation  PCopyOutMin=[]  PCopyOutMax=[]  NCopyOutDataTypeStr=Inherit: Inherit via back propagation  NCopyOutMin=[]  NCopyOutMax=[]  IntegratorContinuousStateAttributes=''  IntegratorStateMustResolveToSignalObject=off  IntegratorRTWStateStorageClass=Auto  FilterContinuousStateAttributes=''  FilterStateMustResolveToSignalObject=off  FilterRTWStateStorageClass=Auto  ParallelPVariant=Passthrough  IdealPVariant=InternalParameters  IVariant=InternalParameters  DVariant=Disabled  bVariant=InternalParameters  cVariant=Disabled  IntegratorVariant=Discrete  SatVariant=Enabled  AWVariant=Passthrough  PCopyVariant=Disabled  TRVariant=Disabled  FdbkBlocksVariant=Forward  IdealPFdbkVariant=Disabled  SatFdbkVariant=Disabled  DerivativeFilterVariant=Disabled  NVariant=Disabled  NCopyVariant=Disabled_SignalSpec  FilterICVariant=Disabled  IntegratorICVariant=InternalICs  ExternalResetVariant=Disabled  TRSumVariant=Passthrough  SumFdbkVariant=Disabled  SumVariant=Sum_PI  TsampFilterVariant=InternalTs  TsampNgainVariant=Passthrough  TsampIntegralVariant=Disabled_SignalSpec  ExternalSaturationOutDataTypeStr=Inherit: Same as second input
  PID Controller (2DOF)2 : slpidlib/PID Controller (2DOF)  Controller=PI  Form=Ideal  TimeDomain=Discrete-time  UseExternalTs=off  SampleTime=0.000001  IntegratorMethod=Forward Euler  FilterMethod=Forward Euler  ControllerParametersSource=internal  P=Kpc_2  I=Kic_2  UseKiTs=off  D=0  N=100  UseFilter=on  b=1  c=1  TunerSelectOption=Transfer Function Based (PID Tuner App)  InitialConditionSource=internal  InitialConditionForIntegrator=0  InitialConditionForFilter=0  DifferentiatorICPrevScaledInput=0  ExternalReset=none  TrackingMode=off  Kt=1  LimitOutput=on  SatLimitsSource=internal  UpperSaturationLimit=72/sqrt(3)  LowerSaturationLimit=-72/sqrt(3)  LinearizeAsGain=on  AntiWindupMode=none  Kb=1  LimitIntegrator=off  UpperIntegratorSaturationLimit=inf  LowerIntegratorSaturationLimit=-inf  POutMin=[]  POutMax=[]  IOutMin=[]  IOutMax=[]  DOutMin=[]  DOutMax=[]  NOutMin=[]  NOutMax=[]  bOutMin=[]  bOutMax=[]  cOutMin=[]  cOutMax=[]  SumOutMin=[]  SumOutMax=[]  SaturationOutMin=[]  SaturationOutMax=[]  PParamMin=[]  PParamMax=[]  IParamMin=[]  IParamMax=[]  DParamMin=[]  DParamMax=[]  NParamMin=[]  NParamMax=[]  bParamMin=[]  bParamMax=[]  cParamMin=[]  cParamMax=[]  KbParamMin=[]  KbParamMax=[]  KtParamMin=[]  KtParamMax=[]  KbOutMin=[]  KbOutMax=[]  KtOutMin=[]  KtOutMax=[]  IntegratorOutMin=[]  IntegratorOutMax=[]  FilterOutMin=[]  FilterOutMax=[]  SumI1OutMin=[]  SumI1OutMax=[]  SumI2OutMin=[]  SumI2OutMax=[]  SumI3OutMin=[]  SumI3OutMax=[]  SumI4OutMin=[]  SumI4OutMax=[]  SumDOutMin=[]  SumDOutMax=[]  Sum1OutMin=[]  Sum1OutMax=[]  Sum2OutMin=[]  Sum2OutMax=[]  Sum3OutMin=[]  Sum3OutMax=[]  DifferentiatorOutMin=[]  DifferentiatorOutMax=[]  FilterDiffOutCoefMin=[]  FilterDiffOutCoefMax=[]  ReciprocalOutMin=[]  ReciprocalOutMax=[]  SumDenOutMin=[]  SumDenOutMax=[]  SumNumOutMin=[]  SumNumOutMax=[]  DivideOutMin=[]  DivideOutMax=[]  UdiffTsProdOutMin=[]  UdiffTsProdOutMax=[]  NTsProdOutMin=[]  NTsProdOutMax=[]  UintegralTsProdOutMin=[]  UintegralTsProdOutMax=[]  UngainTsProdOutMin=[]  UngainTsProdOutMax=[]  ClampingZeroOutDataTypeStr=Inherit: Inherit via back propagation  ClampingZeroOutMin=[]  ClampingZeroOutMax=[]  FilterDenConstantOutDataTypeStr=Inherit: Inherit via back propagation  FilterDenConstantOutMin=[]  FilterDenConstantOutMax=[]  PCopyOutDataTypeStr=Inherit: Inherit via back propagation  PCopyOutMin=[]  PCopyOutMax=[]  NCopyOutDataTypeStr=Inherit: Inherit via back propagation  NCopyOutMin=[]  NCopyOutMax=[]  IntegratorContinuousStateAttributes=''  IntegratorStateMustResolveToSignalObject=off  IntegratorRTWStateStorageClass=Auto  FilterContinuousStateAttributes=''  FilterStateMustResolveToSignalObject=off  FilterRTWStateStorageClass=Auto  ParallelPVariant=Passthrough  IdealPVariant=InternalParameters  IVariant=InternalParameters  DVariant=Disabled  bVariant=InternalParameters  cVariant=Disabled  IntegratorVariant=Discrete  SatVariant=Enabled  AWVariant=Passthrough  PCopyVariant=Disabled  TRVariant=Disabled  FdbkBlocksVariant=Forward  IdealPFdbkVariant=Disabled  SatFdbkVariant=Disabled  DerivativeFilterVariant=Disabled  NVariant=Disabled  NCopyVariant=Disabled_SignalSpec  FilterICVariant=Disabled  IntegratorICVariant=InternalICs  ExternalResetVariant=Disabled  TRSumVariant=Passthrough  SumFdbkVariant=Disabled  SumVariant=Sum_PI  TsampFilterVariant=InternalTs  TsampNgainVariant=Passthrough  TsampIntegralVariant=Disabled_SignalSpec  ExternalSaturationOutDataTypeStr=Inherit: Same as second input
  Sum : Sum  Inputs=|++
  ud_equation : Outport
  uq_equation : Outport  Port=2
  wires:
  PID Controller (2DOF)1/1 -> uq_equation/1
  id/1 -> PID Controller (2DOF)2/2
  iq/1 -> PID Controller (2DOF)1/2
  Constant2/1 -> PID Controller (2DOF)2/1
  PID Controller (2DOF)2/1 -> ud_equation/1
  i_ref/1 -> Sum/1
  Sum/1 -> PID Controller (2DOF)1/1
  Tdisturb/Kt/1 -> Sum/2

== system Control/优化关节模型+电压前馈解耦+PI控制器参数设计+力矩补偿1/速度环PI控制器 ==
  note: rad/s
  note: rpm
  w_mref : Inport
  wm : Inport  Port=2
  Gain3 : Gain  Gain=NtoW
  PID Controller (2DOF)7 : slpidlib/PID Controller (2DOF)  Controller=PI  Form=Ideal  TimeDomain=Discrete-time  UseExternalTs=off  SampleTime=0.000001  IntegratorMethod=Forward Euler  FilterMethod=Forward Euler  ControllerParametersSource=internal  P=Kps_2  I=Kis_2  UseKiTs=off  D=0  N=100  UseFilter=on  b=1  c=1  TunerSelectOption=Transfer Function Based (PID Tuner App)  InitialConditionSource=internal  InitialConditionForIntegrator=0  InitialConditionForFilter=0  DifferentiatorICPrevScaledInput=0  ExternalReset=none  TrackingMode=off  Kt=1  LimitOutput=on  SatLimitsSource=internal  UpperSaturationLimit=23  LowerSaturationLimit=-23  LinearizeAsGain=on  AntiWindupMode=none  Kb=1  LimitIntegrator=off  UpperIntegratorSaturationLimit=inf  LowerIntegratorSaturationLimit=-inf  POutMin=[]  POutMax=[]  IOutMin=[]  IOutMax=[]  DOutMin=[]  DOutMax=[]  NOutMin=[]  NOutMax=[]  bOutMin=[]  bOutMax=[]  cOutMin=[]  cOutMax=[]  SumOutMin=[]  SumOutMax=[]  SaturationOutMin=[]  SaturationOutMax=[]  PParamMin=[]  PParamMax=[]  IParamMin=[]  IParamMax=[]  DParamMin=[]  DParamMax=[]  NParamMin=[]  NParamMax=[]  bParamMin=[]  bParamMax=[]  cParamMin=[]  cParamMax=[]  KbParamMin=[]  KbParamMax=[]  KtParamMin=[]  KtParamMax=[]  KbOutMin=[]  KbOutMax=[]  KtOutMin=[]  KtOutMax=[]  IntegratorOutMin=[]  IntegratorOutMax=[]  FilterOutMin=[]  FilterOutMax=[]  SumI1OutMin=[]  SumI1OutMax=[]  SumI2OutMin=[]  SumI2OutMax=[]  SumI3OutMin=[]  SumI3OutMax=[]  SumI4OutMin=[]  SumI4OutMax=[]  SumDOutMin=[]  SumDOutMax=[]  Sum1OutMin=[]  Sum1OutMax=[]  Sum2OutMin=[]  Sum2OutMax=[]  Sum3OutMin=[]  Sum3OutMax=[]  DifferentiatorOutMin=[]  DifferentiatorOutMax=[]  FilterDiffOutCoefMin=[]  FilterDiffOutCoefMax=[]  ReciprocalOutMin=[]  ReciprocalOutMax=[]  SumDenOutMin=[]  SumDenOutMax=[]  SumNumOutMin=[]  SumNumOutMax=[]  DivideOutMin=[]  DivideOutMax=[]  UdiffTsProdOutMin=[]  UdiffTsProdOutMax=[]  NTsProdOutMin=[]  NTsProdOutMax=[]  UintegralTsProdOutMin=[]  UintegralTsProdOutMax=[]  UngainTsProdOutMin=[]  UngainTsProdOutMax=[]  ClampingZeroOutDataTypeStr=Inherit: Inherit via back propagation  ClampingZeroOutMin=[]  ClampingZeroOutMax=[]  FilterDenConstantOutDataTypeStr=Inherit: Inherit via back propagation  FilterDenConstantOutMin=[]  FilterDenConstantOutMax=[]  PCopyOutDataTypeStr=Inherit: Inherit via back propagation  PCopyOutMin=[]  PCopyOutMax=[]  NCopyOutDataTypeStr=Inherit: Inherit via back propagation  NCopyOutMin=[]  NCopyOutMax=[]  IntegratorContinuousStateAttributes=''  IntegratorStateMustResolveToSignalObject=off  IntegratorRTWStateStorageClass=Auto  FilterContinuousStateAttributes=''  FilterStateMustResolveToSignalObject=off  FilterRTWStateStorageClass=Auto  ParallelPVariant=Passthrough  IdealPVariant=InternalParameters  IVariant=InternalParameters  DVariant=Disabled  bVariant=InternalParameters  cVariant=Disabled  IntegratorVariant=Discrete  SatVariant=Enabled  AWVariant=Passthrough  PCopyVariant=Disabled  TRVariant=Disabled  FdbkBlocksVariant=Forward  IdealPFdbkVariant=Disabled  SatFdbkVariant=Disabled  DerivativeFilterVariant=Disabled  NVariant=Disabled  NCopyVariant=Disabled_SignalSpec  FilterICVariant=Disabled  IntegratorICVariant=InternalICs  ExternalResetVariant=Disabled  TRSumVariant=Passthrough  SumFdbkVariant=Disabled  SumVariant=Sum_PI  TsampFilterVariant=InternalTs  TsampNgainVariant=Passthrough  TsampIntegralVariant=Disabled_SignalSpec  ExternalSaturationOutDataTypeStr=Inherit: Same as second input
  i_ref : Outport
  wires:
  w_mref/1 -> Gain3/1
  PID Controller (2DOF)7/1 -> i_ref/1
  wm/1 -> PID Controller (2DOF)7/2
  Gain3/1 -> PID Controller (2DOF)7/1

== system Control/优化关节模型+电压前馈解耦+PI控制器参数设计1/Inverter ==
  Pluse : Inport
  DC Voltage Source1 : spsDCVoltageSourceLib/DC Voltage Source  Amplitude=U_dc  Measurements=None
  Universal Bridge : spsUniversalBridgeLib/Universal Bridge  Arms=3  SnubberResistance=1e5  SnubberCapacitance=inf  Device=IGBT / Diodes  Ron=1e-3  Lon=0  ForwardVoltages="[  0  0  ]"  ForwardVoltage=0  GTOparameters=[ 10e-6 , 20e-6 ]  IGBTparameters=[ 1e-6 , 2e-6 ]  Measurements=None  Measurements_2=None  converterType=Rectifier
  A : PMIOPort  Side=Right
  B : PMIOPort  Port=2  Side=Right
  C : PMIOPort  Port=3  Side=Right
  wires:
  Pluse/1 -> Universal Bridge/1
  connections:
  Universal Bridge/LConn1 -- A/RConn1
  Universal Bridge/LConn3 -- C/RConn1
  DC Voltage Source1/LConn1 -- Universal Bridge/RConn2
  DC Voltage Source1/RConn1 -- Universal Bridge/RConn1
  Universal Bridge/LConn2 -- B/RConn1

== system Control/优化关节模型+电压前馈解耦+PI控制器参数设计1/Joint ==
  w_m : Inport
  TL : Inport  Port=2
  Permanent Magnet Synchronous Machine : spsPermanentMagnetSynchronousMachineLib/Permanent Magnet Synchronous Machine  NbPhases=3  FluxDistribution=Sinusoidal  RotorType=Round  MechanicalLoad=Torque Tm  PresetModel=No  ShowDetailedParameters=on  MeasurementBus=off  Resistance=R_s  Inductance=8.5e-3  dqInductances=[2.27e-3,2.045e-3]  La=L_q  MachineConstant=Torque Constant (N.m / A_peak)  Flux=0.01337  VoltageCst=33.9507  TorqueCst=K_t  Flat=120  Mechanical=[J_total 0 P_n 0]  PolePairs=4  InitialConditions=[0,0, 0,0]  InitialConditions5ph=[0 0 0 0 0 0]  RefAngle=Aligned with phase A axis (original Park)  IterativeDiscreteModel=Trapezoidal non iterative  TsBlock=-1  TsPowergui=0
  Subsystem : Subsystem
  A : PMIOPort  Side=Left
  B : PMIOPort  Port=2  Side=Left
  C : PMIOPort  Port=3  Side=Left
  m : Outport
  wires:
  w_m/1 -> Subsystem/1(wm)
  Subsystem/1(Tm) -> Permanent Magnet Synchronous Machine/1
  Permanent Magnet Synchronous Machine/1 -> m/1
  TL/1 -> Subsystem/2(TL)
  connections:
  C/RConn1 -- Permanent Magnet Synchronous Machine/LConn3
  B/RConn1 -- Permanent Magnet Synchronous Machine/LConn2
  A/RConn1 -- Permanent Magnet Synchronous Machine/LConn1

== system Control/优化关节模型+电压前馈解耦+PI控制器参数设计1/SVPWM1 ==
  Uα : Inport
  Uβ : Inport  Port=2
  SVPWM Generator (2-Level) : spsSVPWMGenerator2LevelLib/SVPWM Generator (2-Level)  InputType=alpha-beta components  SwitchingPattern=Pattern #1  Fc=1/TPWM  ParUref=[0.8 -30 50]  Ts=0.000001
  Pulse : Outport
  wires:
  Uβ/1 -> SVPWM Generator (2-Level)/2
  Uα/1 -> SVPWM Generator (2-Level)/1
  SVPWM Generator (2-Level)/1 -> Pulse/1

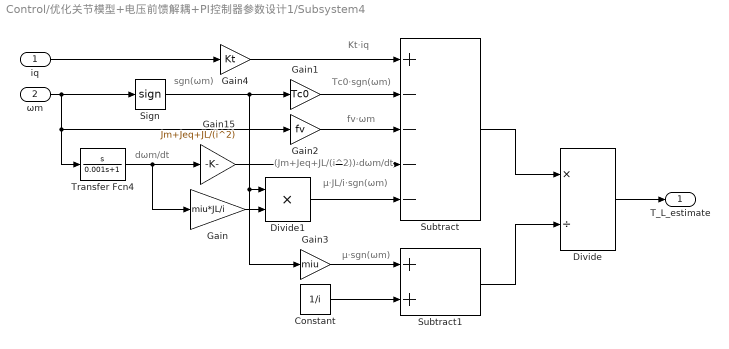
== system Control/优化关节模型+电压前馈解耦+PI控制器参数设计1/Subsystem4 ==
  note: fv·ωm
  note: (Jm+Jeq+JL/(i^2))·dωm/dt
  note: Kt·iq
  note: Tc0·sgn(ωm)
  note: dωm/dt
  note: sgn(ωm)
  note: μ·JL/i·sgn(ωm)
  note: μ·sgn(ωm)
  iq : Inport
  ωm : Inport  Port=2
  Constant : Constant  Value=1/i
  Divide : Product  Inputs=*/
  Divide1 : Product  Inputs=**
  Gain : Gain  Gain=miu*JL/i
  Gain1 : Gain  Gain=Tc0
  Gain15 : Gain  Gain=Jm+Jeq+JL/(i^2)
  Gain2 : Gain  Gain=fv
  Gain3 : Gain  Gain=miu
  Gain4 : Gain  Gain=Kt
  Sign : Signum
  Subtract : Sum  Inputs=+----
  Subtract1 : Sum
  Transfer Fcn4 : TransferFcn  Numerator=[1 0]  Denominator=[0.001 1]
  T_L_estimate : Outport
  wires:
  Gain4/1 -> Subtract/1
  ωm/1 -> Transfer Fcn4/1, Gain2/1, Sign/1
  Gain15/1 -> Subtract/4
  Divide/1 -> T_L_estimate/1
  Subtract/1 -> Divide/1
  Gain2/1 -> Subtract/3
  Gain1/1 -> Subtract/2
  Sign/1 -> Gain3/1, Divide1/1, Gain1/1
  iq/1 -> Gain4/1
  Constant/1 -> Subtract1/2
  Transfer Fcn4/1 -> Gain15/1, Gain/1
  Gain/1 -> Divide1/2
  Divide1/1 -> Subtract/5
  Gain3/1 -> Subtract1/1
  Subtract1/1 -> Divide/2

== system Control/优化关节模型+电压前馈解耦+PI控制器参数设计1/电压前馈补偿 ==
  w_m : Inport
  iq : Inport  Port=2
  id : Inport  Port=3
  Add : Sum
  Constant2 : Constant  Value=phi_f
  Gain1 : Gain  Gain=L_d
  Gain2 : Gain  Gain=P_n
  Gain7 : Gain  Gain=L_q
  Product : Product
  Product1 : Product
  uq_compensation : Outport
  ud_compensation : Outport  Port=2
  wires:
  w_m/1 -> Gain2/1
  iq/1 -> Product/2
  Gain7/1 -> ud_compensation/1
  Product/1 -> Gain7/1
  Gain1/1 -> Add/1
  Gain2/1 -> Product1/1, Product/1
  Add/1 -> Product1/2
  id/1 -> Gain1/1
  Product1/1 -> uq_compensation/1
  Constant2/1 -> Add/2

== system Control/优化关节模型+电压前馈解耦+PI控制器参数设计1/电流环PI控制器 ==
  note: ud_equation
  note: uq_equation
  i_ref : Inport
  id : Inport  Port=2
  iq : Inport  Port=3
  Constant2 : Constant  Value=0
  PID Controller (2DOF)1 : slpidlib/PID Controller (2DOF)  Controller=PI  Form=Ideal  TimeDomain=Discrete-time  UseExternalTs=off  SampleTime=0.000001  IntegratorMethod=Forward Euler  FilterMethod=Forward Euler  ControllerParametersSource=internal  P=Kpc_2  I=Kic_2  UseKiTs=off  D=0  N=100  UseFilter=on  b=1  c=1  TunerSelectOption=Transfer Function Based (PID Tuner App)  InitialConditionSource=internal  InitialConditionForIntegrator=0  InitialConditionForFilter=0  DifferentiatorICPrevScaledInput=0  ExternalReset=none  TrackingMode=off  Kt=1  LimitOutput=on  SatLimitsSource=internal  UpperSaturationLimit=72/sqrt(3)  LowerSaturationLimit=-72/sqrt(3)  LinearizeAsGain=on  AntiWindupMode=none  Kb=1  LimitIntegrator=off  UpperIntegratorSaturationLimit=inf  LowerIntegratorSaturationLimit=-inf  POutMin=[]  POutMax=[]  IOutMin=[]  IOutMax=[]  DOutMin=[]  DOutMax=[]  NOutMin=[]  NOutMax=[]  bOutMin=[]  bOutMax=[]  cOutMin=[]  cOutMax=[]  SumOutMin=[]  SumOutMax=[]  SaturationOutMin=[]  SaturationOutMax=[]  PParamMin=[]  PParamMax=[]  IParamMin=[]  IParamMax=[]  DParamMin=[]  DParamMax=[]  NParamMin=[]  NParamMax=[]  bParamMin=[]  bParamMax=[]  cParamMin=[]  cParamMax=[]  KbParamMin=[]  KbParamMax=[]  KtParamMin=[]  KtParamMax=[]  KbOutMin=[]  KbOutMax=[]  KtOutMin=[]  KtOutMax=[]  IntegratorOutMin=[]  IntegratorOutMax=[]  FilterOutMin=[]  FilterOutMax=[]  SumI1OutMin=[]  SumI1OutMax=[]  SumI2OutMin=[]  SumI2OutMax=[]  SumI3OutMin=[]  SumI3OutMax=[]  SumI4OutMin=[]  SumI4OutMax=[]  SumDOutMin=[]  SumDOutMax=[]  Sum1OutMin=[]  Sum1OutMax=[]  Sum2OutMin=[]  Sum2OutMax=[]  Sum3OutMin=[]  Sum3OutMax=[]  DifferentiatorOutMin=[]  DifferentiatorOutMax=[]  FilterDiffOutCoefMin=[]  FilterDiffOutCoefMax=[]  ReciprocalOutMin=[]  ReciprocalOutMax=[]  SumDenOutMin=[]  SumDenOutMax=[]  SumNumOutMin=[]  SumNumOutMax=[]  DivideOutMin=[]  DivideOutMax=[]  UdiffTsProdOutMin=[]  UdiffTsProdOutMax=[]  NTsProdOutMin=[]  NTsProdOutMax=[]  UintegralTsProdOutMin=[]  UintegralTsProdOutMax=[]  UngainTsProdOutMin=[]  UngainTsProdOutMax=[]  ClampingZeroOutDataTypeStr=Inherit: Inherit via back propagation  ClampingZeroOutMin=[]  ClampingZeroOutMax=[]  FilterDenConstantOutDataTypeStr=Inherit: Inherit via back propagation  FilterDenConstantOutMin=[]  FilterDenConstantOutMax=[]  PCopyOutDataTypeStr=Inherit: Inherit via back propagation  PCopyOutMin=[]  PCopyOutMax=[]  NCopyOutDataTypeStr=Inherit: Inherit via back propagation  NCopyOutMin=[]  NCopyOutMax=[]  IntegratorContinuousStateAttributes=''  IntegratorStateMustResolveToSignalObject=off  IntegratorRTWStateStorageClass=Auto  FilterContinuousStateAttributes=''  FilterStateMustResolveToSignalObject=off  FilterRTWStateStorageClass=Auto  ParallelPVariant=Passthrough  IdealPVariant=InternalParameters  IVariant=InternalParameters  DVariant=Disabled  bVariant=InternalParameters  cVariant=Disabled  IntegratorVariant=Discrete  SatVariant=Enabled  AWVariant=Passthrough  PCopyVariant=Disabled  TRVariant=Disabled  FdbkBlocksVariant=Forward  IdealPFdbkVariant=Disabled  SatFdbkVariant=Disabled  DerivativeFilterVariant=Disabled  NVariant=Disabled  NCopyVariant=Disabled_SignalSpec  FilterICVariant=Disabled  IntegratorICVariant=InternalICs  ExternalResetVariant=Disabled  TRSumVariant=Passthrough  SumFdbkVariant=Disabled  SumVariant=Sum_PI  TsampFilterVariant=InternalTs  TsampNgainVariant=Passthrough  TsampIntegralVariant=Disabled_SignalSpec  ExternalSaturationOutDataTypeStr=Inherit: Same as second input
  PID Controller (2DOF)2 : slpidlib/PID Controller (2DOF)  Controller=PI  Form=Ideal  TimeDomain=Discrete-time  UseExternalTs=off  SampleTime=0.000001  IntegratorMethod=Forward Euler  FilterMethod=Forward Euler  ControllerParametersSource=internal  P=Kpc_2  I=Kic_2  UseKiTs=off  D=0  N=100  UseFilter=on  b=1  c=1  TunerSelectOption=Transfer Function Based (PID Tuner App)  InitialConditionSource=internal  InitialConditionForIntegrator=0  InitialConditionForFilter=0  DifferentiatorICPrevScaledInput=0  ExternalReset=none  TrackingMode=off  Kt=1  LimitOutput=on  SatLimitsSource=internal  UpperSaturationLimit=72/sqrt(3)  LowerSaturationLimit=-72/sqrt(3)  LinearizeAsGain=on  AntiWindupMode=none  Kb=1  LimitIntegrator=off  UpperIntegratorSaturationLimit=inf  LowerIntegratorSaturationLimit=-inf  POutMin=[]  POutMax=[]  IOutMin=[]  IOutMax=[]  DOutMin=[]  DOutMax=[]  NOutMin=[]  NOutMax=[]  bOutMin=[]  bOutMax=[]  cOutMin=[]  cOutMax=[]  SumOutMin=[]  SumOutMax=[]  SaturationOutMin=[]  SaturationOutMax=[]  PParamMin=[]  PParamMax=[]  IParamMin=[]  IParamMax=[]  DParamMin=[]  DParamMax=[]  NParamMin=[]  NParamMax=[]  bParamMin=[]  bParamMax=[]  cParamMin=[]  cParamMax=[]  KbParamMin=[]  KbParamMax=[]  KtParamMin=[]  KtParamMax=[]  KbOutMin=[]  KbOutMax=[]  KtOutMin=[]  KtOutMax=[]  IntegratorOutMin=[]  IntegratorOutMax=[]  FilterOutMin=[]  FilterOutMax=[]  SumI1OutMin=[]  SumI1OutMax=[]  SumI2OutMin=[]  SumI2OutMax=[]  SumI3OutMin=[]  SumI3OutMax=[]  SumI4OutMin=[]  SumI4OutMax=[]  SumDOutMin=[]  SumDOutMax=[]  Sum1OutMin=[]  Sum1OutMax=[]  Sum2OutMin=[]  Sum2OutMax=[]  Sum3OutMin=[]  Sum3OutMax=[]  DifferentiatorOutMin=[]  DifferentiatorOutMax=[]  FilterDiffOutCoefMin=[]  FilterDiffOutCoefMax=[]  ReciprocalOutMin=[]  ReciprocalOutMax=[]  SumDenOutMin=[]  SumDenOutMax=[]  SumNumOutMin=[]  SumNumOutMax=[]  DivideOutMin=[]  DivideOutMax=[]  UdiffTsProdOutMin=[]  UdiffTsProdOutMax=[]  NTsProdOutMin=[]  NTsProdOutMax=[]  UintegralTsProdOutMin=[]  UintegralTsProdOutMax=[]  UngainTsProdOutMin=[]  UngainTsProdOutMax=[]  ClampingZeroOutDataTypeStr=Inherit: Inherit via back propagation  ClampingZeroOutMin=[]  ClampingZeroOutMax=[]  FilterDenConstantOutDataTypeStr=Inherit: Inherit via back propagation  FilterDenConstantOutMin=[]  FilterDenConstantOutMax=[]  PCopyOutDataTypeStr=Inherit: Inherit via back propagation  PCopyOutMin=[]  PCopyOutMax=[]  NCopyOutDataTypeStr=Inherit: Inherit via back propagation  NCopyOutMin=[]  NCopyOutMax=[]  IntegratorContinuousStateAttributes=''  IntegratorStateMustResolveToSignalObject=off  IntegratorRTWStateStorageClass=Auto  FilterContinuousStateAttributes=''  FilterStateMustResolveToSignalObject=off  FilterRTWStateStorageClass=Auto  ParallelPVariant=Passthrough  IdealPVariant=InternalParameters  IVariant=InternalParameters  DVariant=Disabled  bVariant=InternalParameters  cVariant=Disabled  IntegratorVariant=Discrete  SatVariant=Enabled  AWVariant=Passthrough  PCopyVariant=Disabled  TRVariant=Disabled  FdbkBlocksVariant=Forward  IdealPFdbkVariant=Disabled  SatFdbkVariant=Disabled  DerivativeFilterVariant=Disabled  NVariant=Disabled  NCopyVariant=Disabled_SignalSpec  FilterICVariant=Disabled  IntegratorICVariant=InternalICs  ExternalResetVariant=Disabled  TRSumVariant=Passthrough  SumFdbkVariant=Disabled  SumVariant=Sum_PI  TsampFilterVariant=InternalTs  TsampNgainVariant=Passthrough  TsampIntegralVariant=Disabled_SignalSpec  ExternalSaturationOutDataTypeStr=Inherit: Same as second input
  ud_equation : Outport
  uq_equation : Outport  Port=2
  wires:
  i_ref/1 -> PID Controller (2DOF)1/1
  PID Controller (2DOF)2/1 -> ud_equation/1
  Constant2/1 -> PID Controller (2DOF)2/1
  iq/1 -> PID Controller (2DOF)1/2
  id/1 -> PID Controller (2DOF)2/2
  PID Controller (2DOF)1/1 -> uq_equation/1
